simulink model "CurrentReferenceTest"  (R2026a)
settings: Solver=FixedStepDiscrete  StopTime=refTestCfg.Duration  FixedStep=currentCfg.Ts
PostLoadFcn:
  | addpath(fullfile(fileparts(fileparts(fileparts(fileparts(fileparts(get_param(bdroot,'FileName')))))),'docs','scripts'));initialize_motor_paths();initialize_mtpa_fw_model(bdroot);
model workspace (MAT data in the model file):
  currentCfg.Ts = 0.0001
  currentCfg.BandwidthHz = 500
  currentCfg.Kpd = 3.14159265359
  currentCfg.Kpq = 3.76991118431
  currentCfg.Kid = 1570.79632679
  currentCfg.Kiq = 1570.79632679
  currentCfg.Kaw = 1000
  deadtimeCfg.DeadTime = 2e-06
  deadtimeCfg.DeviceDrop = 0
  deadtimeCfg.CurrentBlend = 0.1
  deadtimeCfg.ModelEnable = 0
  deadtimeCfg.CompensationEnable = 0
  deadtimeCfg.CompensationScale = 1
  deadtimeCfg.SwitchingStep = 1e-07
  experimentCfg.Step = 5e-06
  experimentCfg.LogTs = 0.0001
  experimentCfg.Duration = 1.5
  experimentCfg.Mode = 2
  experimentCfg.UseInverter = 1
  experimentCfg.UseTiming = 1
  experimentCfg.UseMechanical = 1
  experimentCfg.ImposedElectricalSpeed = 0
  experimentCfg.IdReference = 0
  experimentCfg.IqReference = 2
  experimentCfg.IqInitial = 0
  experimentCfg.SpeedReference = 40
  experimentCfg.SpeedInitial = 0
  experimentCfg.PositionReference = 1
  experimentCfg.PositionInitial = 0
  experimentCfg.CommandTime = 0.05
  experimentCfg.LoadTorque = 0.1
  experimentCfg.LoadTime = 0.35
  experimentCfg.Enable = 1
  experimentCfg.Reset = 0
  feedforwardCfg.Enable = 0
  feedforwardCfg.ParameterScale = 1
  inverterCfg.Vdc = 48
  inverterCfg.MinDuty = 0.02
  inverterCfg.PwmTs = 0.0001
  inverterCfg.LinearLimit = 26.6043004043
  motionCfg.Ts = 0.001
  motionCfg.NaturalFrequency = 20
  motionCfg.Damping = 0.9
  motionCfg.Kt = 0.21
  motionCfg.Kp = 0.0852380952381
  motionCfg.Ki = 0.952380952381
  motionCfg.Kaw = 20
  motionCfg.PositionKp = 8
  motionCfg.SpeedLimit = 80
  motionCfg.AccelerationLimit = 200
  motionCfg.CurrentLimit = 8
  pmsmCfg.Rs = 0.5
  pmsmCfg.Ld = 0.001
  pmsmCfg.Lq = 0.0012
  pmsmCfg.Flux = 0.035
  pmsmCfg.PolePairs = 4
  pmsmCfg.J = 0.0005
  pmsmCfg.B = 0.0001
  pmsmCfg.Id0 = 0
  pmsmCfg.Iq0 = 0
  pmsmCfg.Speed0 = 0
  pmsmCfg.Position0 = 0
  refCfg.MtpaEnable = 1
  refCfg.FwEnable = 1
  refCfg.CurrentMax = 8
  refCfg.IdMin = -7
  refCfg.VoltageReserve = 0.95
  refCfg.FwVoltageMargin = 0.2
  refCfg.MinDuty = 0.02
  refCfg.FwTs = 0.001
  refCfg.FilterTau = 0.003
  refCfg.FwKi = 50
  refCfg.IdSlew = 200
  refCfg.TablePoints = 257
  refCfg.SpeedTs = 0.001
  refCfg.SpeedKp = 0.0179
  refCfg.SpeedKi = 0.2
  refCfg.SpeedKaw = 20
  refCfg.IdTable = [0 -5.58035678697e-06 -2.23214228772e-05 -5.02231854586e-05 -8.9285623178e-05 -0.000139508706141 -0.000200892395911 -0.000273436645513 -0.000357141399429 -0.0004520065936 -0.00055803215543 -0.000675218003779 ... (257 elements, 1x257)]
  refCfg.TorqueGrid = [0 0.00656250010463 0.0131250008371 0.0196875028251 0.0262500066964 0.0328125130789 0.0393750226004 0.0459375358886 0.0525000535713 0.0590625762763 0.0656251046313 0.0721876392641 ... (257 elements, 1x257)]
  refCfg.MaxTorque = 1.68175087053
  refCfg.Kt = 0.21
  refCfg.VoltageFactor = 0.526543445501
  refCfg.FilterAlpha = 0.75
  refTestCfg.Duration = 0.25
  refTestCfg.TorqueReference = 0.2
  refTestCfg.TorqueInitial = 0
  refTestCfg.ElectricalSpeed = 800
  refTestCfg.Vdc = 48
  refTestCfg.VoltageDemand = 28
  testStim.time = []
  testStim.signals.values = [0.2 0.2 0.2 0.2 0.2 0.2 0.2 0.2 0.2 0.2 0.2 0.2 ... (15006 elements, 2501x6)]
  testStim.signals.dimensions = 6
  timingCfg.Ts = 0.0001
  timingCfg.FeedbackTicks = 1
  timingCfg.ActuationTicks = 1
libraries: CurrentReference x1
settings Model: Creator=24322  LastModifiedBy=24322

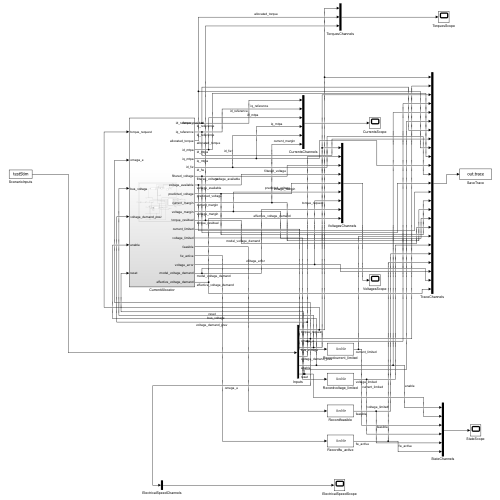
[thumbnail: Simulink's stored preview of the top-level diagram]
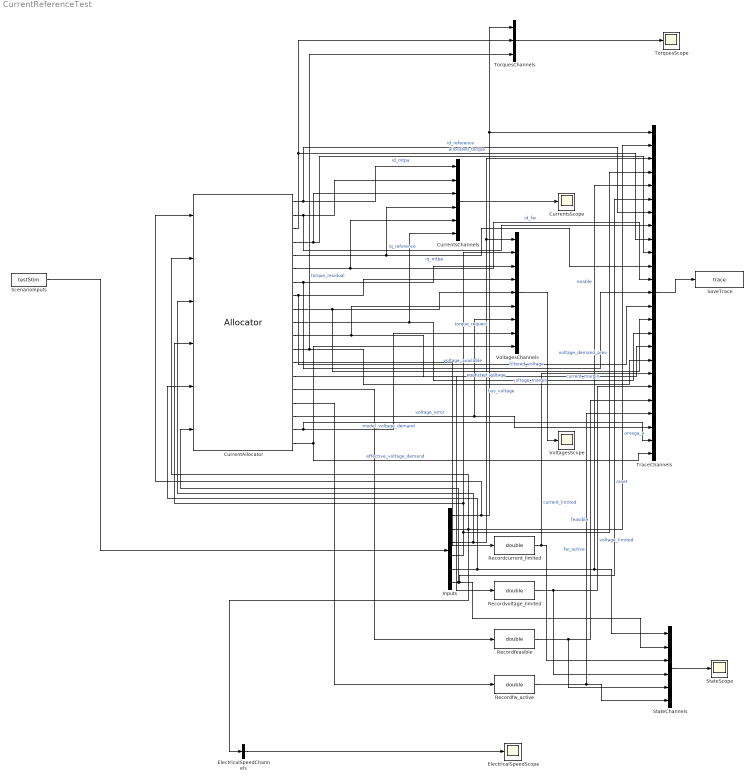
== system CurrentReferenceTest ==
  CurrentAllocator : CurrentReference/Allocator  SystemSampleTime=-1  VariantActivationTime=update diagram  EmptyChoice=off  PassThrough=off  PassThroughVariantControl=(default)  EmptyChoiceVariantControl=(default)  AllowFlexibleInterface=on  Latency=0  AutoFrameSizeCalculation=off
  CurrentsChannels : Mux  Inputs=6
  CurrentsScope : Scope
      settings: Title=Currents  YLabel=A
  ElectricalSpeedChannels : Mux  Inputs=1
  ElectricalSpeedScope : Scope
      settings: Title=ElectricalSpeed  YLabel=rad/s
  Inputs : Demux  Outputs=6
  Recordcurrent_limited : DataTypeConversion  OutDataTypeStr=double  SaturateOnIntegerOverflow=off  RndMeth=Floor
  Recordfeasible : DataTypeConversion  OutDataTypeStr=double  SaturateOnIntegerOverflow=off  RndMeth=Floor
  Recordfw_active : DataTypeConversion  OutDataTypeStr=double  SaturateOnIntegerOverflow=off  RndMeth=Floor
  Recordvoltage_limited : DataTypeConversion  OutDataTypeStr=double  SaturateOnIntegerOverflow=off  RndMeth=Floor
  SaveTrace : ToWorkspace  VariableName=trace  SaveFormat=Structure With Time  SampleTime=currentCfg.Ts
  ScenarioInputs : FromWorkspace  VariableName=testStim  SampleTime=currentCfg.Ts  Interpolate=off  OutputAfterFinalValue=Holding final value
  StateChannels : Mux  Inputs=6
  StateScope : Scope
      settings: Title=State  YLabel=1
  TorquesChannels : Mux  Inputs=3
  TorquesScope : Scope
      settings: Title=Torques  YLabel=N*m
  TraceChannels : Mux  Inputs=25
  VoltagesChannels : Mux  Inputs=9
  VoltagesScope : Scope
      settings: Title=Voltages  YLabel=V
  wires:
  StateChannels/1 -> StateScope/1
  ElectricalSpeedChannels/1 -> ElectricalSpeedScope/1
  TorquesChannels/1 -> TorquesScope/1
  CurrentAllocator/16 -> Recordfw_active/1
  CurrentAllocator/15 -> Recordfeasible/1
  CurrentAllocator/14 -> Recordvoltage_limited/1
  CurrentAllocator/13 -> Recordcurrent_limited/1
  CurrentAllocator/19 -> VoltagesChannels/9, TraceChannels/25  "effective_voltage_demand"
  CurrentAllocator/18 -> VoltagesChannels/8, TraceChannels/24  "model_voltage_demand"
  Inputs/6 -> StateChannels/2, TraceChannels/6, CurrentAllocator/6  "reset"
  Inputs/5 -> StateChannels/1, TraceChannels/5, CurrentAllocator/5  "enable"
  Inputs/4 -> CurrentAllocator/4, VoltagesChannels/2, TraceChannels/4  "voltage_demand_prev"
  Inputs/3 -> VoltagesChannels/1, TraceChannels/3, CurrentAllocator/3  "bus_voltage"
  Inputs/2 -> ElectricalSpeedChannels/1, TraceChannels/2, CurrentAllocator/2  "omega_e"
  Inputs/1 -> TraceChannels/1, TorquesChannels/1, CurrentAllocator/1  "torque_request"
  ScenarioInputs/1 -> Inputs/1
  TraceChannels/1 -> SaveTrace/1
  CurrentAllocator/1 -> CurrentsChannels/1, TraceChannels/7  "id_reference"
  CurrentAllocator/2 -> CurrentsChannels/2, TraceChannels/8  "iq_reference"
  CurrentAllocator/3 -> TorquesChannels/2, TraceChannels/9  "allocated_torque"
  CurrentAllocator/4 -> CurrentsChannels/3, TraceChannels/10  "id_mtpa"
  CurrentAllocator/5 -> CurrentsChannels/4, TraceChannels/11  "iq_mtpa"
  CurrentAllocator/6 -> CurrentsChannels/5, TraceChannels/12  "id_fw"
  CurrentAllocator/7 -> VoltagesChannels/3, TraceChannels/13  "filtered_voltage"
  CurrentAllocator/8 -> VoltagesChannels/4, TraceChannels/14  "voltage_available"
  CurrentAllocator/9 -> VoltagesChannels/5, TraceChannels/15  "predicted_voltage"
  CurrentAllocator/10 -> CurrentsChannels/6, TraceChannels/16  "current_margin"
  CurrentAllocator/11 -> VoltagesChannels/6, TraceChannels/17  "voltage_margin"
  CurrentAllocator/12 -> TorquesChannels/3, TraceChannels/18  "torque_residual"
  Recordcurrent_limited/1 -> StateChannels/3, TraceChannels/19  "current_limited"
  Recordvoltage_limited/1 -> StateChannels/4, TraceChannels/20  "voltage_limited"
  Recordfeasible/1 -> StateChannels/5, TraceChannels/21  "feasible"
  Recordfw_active/1 -> StateChannels/6, TraceChannels/22  "fw_active"
  CurrentAllocator/17 -> VoltagesChannels/7, TraceChannels/23  "voltage_error"
  CurrentsChannels/1 -> CurrentsScope/1
  VoltagesChannels/1 -> VoltagesScope/1
